simulink subsystem "Robot_Control_sub"  (R2026a)
settings: Solver=VariableStepAuto
undefined symbols (not defined in the file): Rebuilt_Hood_Servo_Pos_Max, Rebuilt_Hood_Servo_Pos_Min, TEST_Desired_Hood_Enable_OV, TEST_Desired_Hood_Pos_OV, TEST_Desired_Shooter_FF_DC_OV, TEST_Desired_Shooter_Speed_OV, TEST_Feeder_Motor_DC_OV, TEST_Intake_Arm_Motor_DC_OV, TEST_Intake_Roller_Motor_DC_OV, TEST_Output_Override_Flag, TEST_Transfer_Motor_DC_OV
libraries: Autonomous_lib x1, Disabled_lib x1, Controls_Components_lib x1, Teleop_lib x1, Test_lib x1
(part 2 of 2)

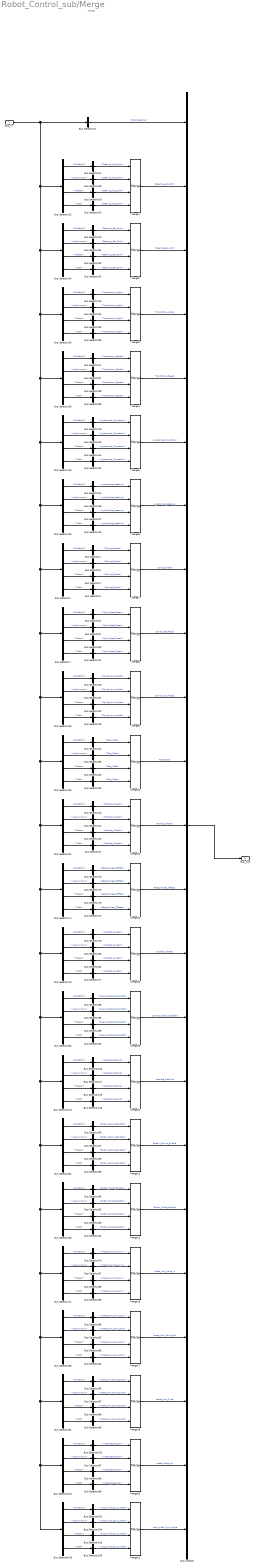
== system Robot_Control_sub/Merge ==
  note: Merge
  Bus_In : Inport
  Bus Creator : BusCreator  Inputs=23
  Bus Selector{1,3..5} (4 alike) : BusSelector  OutputSignals=Spline_Enable
  Bus Selector{9..10,22..23} (4 alike) : BusSelector  OutputSignals=Enable_Wheels
  Bus Selector{97..100} (4 alike) : BusSelector  OutputSignals=Intake_Roller_On
  Bus Selector{2,7,12,14,16,18,20..21,25,50,55,61,66,71,74,79,86,91,94,101,103,121} (22 alike) : BusSelector  OutputSignals=Disabled,Autonomous,Teleop,Test
  Bus Selector{102,104..106} (4 alike) : BusSelector  OutputSignals=Auto_Initial_Gyro_Angle
  Bus Selector{11,28..30} (4 alike) : BusSelector  OutputSignals=Steering_Abs_Cmd
  Bus Selector{117..120} (4 alike) : BusSelector  OutputSignals=Desired_Pipeline
  Bus Selector{13,31..33} (4 alike) : BusSelector  OutputSignals=Steering_Rel_Cmd
  Bus Selector{15,34..36} (4 alike) : BusSelector  OutputSignals=Translation_Angle
  Bus Selector{17,37..39} (4 alike) : BusSelector  OutputSignals=Translation_Speed
  Bus Selector{19,43..45} (4 alike) : BusSelector  OutputSignals=Is_Absolute_Translation
  Bus Selector{24,26..27,46} (4 alike) : BusSelector  OutputSignals=Is_Absolute_Steering
  Bus Selector{6,8,40..41} (4 alike) : BusSelector  OutputSignals=Spline_Ref_Poses
  Bus Selector{42,48..49,51} (4 alike) : BusSelector  OutputSignals=Spline_Num_Poses
  Bus Selector47 : BusSelector  OutputSignals=PreProcessing
  Bus Selector{52..54,56} (4 alike) : BusSelector  OutputSignals=Test_Mode
  Bus Selector{57..60} (4 alike) : BusSelector  OutputSignals=Button_Spinup_Enable
  Bus Selector{62..65} (4 alike) : BusSelector  OutputSignals=Button_Shoot_Enable
  Bus Selector{67..70} (4 alike) : BusSelector  OutputSignals=Intake_Arm_Move_In
  Bus Selector{72..73,75..76} (4 alike) : BusSelector  OutputSignals=Reset_Wheel_Offsets
  Bus Selector{77..78,80..81} (4 alike) : BusSelector  OutputSignals=Disable_Wheels
  Bus Selector{82..85} (4 alike) : BusSelector  OutputSignals=Intake_Arm_Move_Out
  Bus Selector{87..90} (4 alike) : BusSelector  OutputSignals=Intake_Arm_Move_Cycle
  Bus Selector{92..93,95..96} (4 alike) : BusSelector  OutputSignals=Swerve_Motors_Disabled
  Merge{1..21,24} (22 alike) : Merge  Inputs=4
  Bus_Out : Outport
  wires:
  Bus_In/1 -> Bus Selector47/1, Bus Selector12/1, Bus Selector14/1, Bus Selector16/1, Bus Selector18/1, Bus Selector20/1, Bus Selector25/1, Bus Selector21/1, Bus Selector74/1, Bus Selector121/1, Bus Selector61/1, Bus Selector66/1, Bus Selector71/1, Bus Selector86/1, Bus Selector91/1, Bus Selector101/1, Bus Selector103/1, Bus Selector94/1, Bus Selector79/1, Bus Selector55/1, Bus Selector50/1, Bus Selector7/1, Bus Selector2/1
  Merge21/1 -> Bus Creator/23  "Auto_Initial_Gyro_Angle"
  Bus Selector103/2 -> Bus Selector104/1  "<Autonomous>"
  Bus Selector105/1 -> Merge21/3  "<Auto_Initial_Gyro_Angle>"
  Bus Selector103/3 -> Bus Selector105/1  "<Teleop>"
  Bus Selector102/1 -> Merge21/1  "<Auto_Initial_Gyro_Angle>"
  Bus Selector104/1 -> Merge21/2  "<Auto_Initial_Gyro_Angle>"
  Bus Selector103/1 -> Bus Selector102/1  "<Disabled>"
  Bus Selector103/4 -> Bus Selector106/1  "<Test>"
  Bus Selector106/1 -> Merge21/4  "<Auto_Initial_Gyro_Angle>"
  Bus Selector99/1 -> Merge20/4  "<Intake_Roller_On>"
  Bus Selector98/1 -> Merge20/3  "<Intake_Roller_On>"
  Bus Selector97/1 -> Merge20/2  "<Intake_Roller_On>"
  Bus Selector89/1 -> Merge18/4  "<Intake_Arm_Move_Cycle>"
  Bus Selector88/1 -> Merge18/3  "<Intake_Arm_Move_Cycle>"
  Bus Selector87/1 -> Merge18/2  "<Intake_Arm_Move_Cycle>"
  Bus Selector84/1 -> Merge17/4  "<Intake_Arm_Move_Out>"
  Bus Selector83/1 -> Merge17/3  "<Intake_Arm_Move_Out>"
  Bus Selector82/1 -> Merge17/2  "<Intake_Arm_Move_Out>"
  Bus Selector69/1 -> Merge13/4  "<Intake_Arm_Move_In>"
  Bus Selector68/1 -> Merge13/3  "<Intake_Arm_Move_In>"
  Bus Selector67/1 -> Merge13/2  "<Intake_Arm_Move_In>"
  Merge20/1 -> Bus Creator/22  "Intake_Roller_On"
  Bus Selector101/1 -> Bus Selector100/1  "<Disabled>"
  Bus Selector101/3 -> Bus Selector98/1  "<Teleop>"
  Bus Selector100/1 -> Merge20/1  "<Intake_Roller_On>"
  Bus Selector101/2 -> Bus Selector97/1  "<Autonomous>"
  Bus Selector101/4 -> Bus Selector99/1  "<Test>"
  Merge18/1 -> Bus Creator/21  "Intake_Arm_Cycle"
  Bus Selector91/4 -> Bus Selector89/1  "<Test>"
  Bus Selector91/2 -> Bus Selector87/1  "<Autonomous>"
  Bus Selector90/1 -> Merge18/1  "<Intake_Arm_Move_Cycle>"
  Bus Selector91/3 -> Bus Selector88/1  "<Teleop>"
  Bus Selector91/1 -> Bus Selector90/1  "<Disabled>"
  Merge17/1 -> Bus Creator/20  "Intake_Arm_Move_Out"
  Bus Selector86/1 -> Bus Selector85/1  "<Disabled>"
  Bus Selector86/3 -> Bus Selector83/1  "<Teleop>"
  Bus Selector85/1 -> Merge17/1  "<Intake_Arm_Move_Out>"
  Bus Selector86/2 -> Bus Selector82/1  "<Autonomous>"
  Bus Selector86/4 -> Bus Selector84/1  "<Test>"
  Merge13/1 -> Bus Creator/19  "Intake_Arm_Move_In"
  Bus Selector71/4 -> Bus Selector69/1  "<Test>"
  Bus Selector70/1 -> Merge13/1  "<Intake_Arm_Move_In>"
  Bus Selector71/1 -> Bus Selector70/1  "<Disabled>"
  Bus Selector71/3 -> Bus Selector68/1  "<Teleop>"
  Bus Selector71/2 -> Bus Selector67/1  "<Autonomous>"
  Bus Selector64/1 -> Merge12/4  "<Button_Shoot_Enable>"
  Bus Selector63/1 -> Merge12/3  "<Button_Shoot_Enable>"
  Bus Selector62/1 -> Merge12/2  "<Button_Shoot_Enable>"
  Bus Selector59/1 -> Merge11/4  "<Button_Spinup_Enable>"
  Bus Selector58/1 -> Merge11/3  "<Button_Spinup_Enable>"
  Bus Selector57/1 -> Merge11/2  "<Button_Spinup_Enable>"
  Bus Selector65/1 -> Merge12/1  "<Button_Shoot_Enable>"
  Bus Selector66/2 -> Bus Selector62/1  "<Autonomous>"
  Bus Selector66/3 -> Bus Selector63/1  "<Teleop>"
  Bus Selector66/1 -> Bus Selector65/1  "<Disabled>"
  Bus Selector66/4 -> Bus Selector64/1  "<Test>"
  Bus Selector61/2 -> Bus Selector57/1  "<Autonomous>"
  Bus Selector60/1 -> Merge11/1  "<Button_Spinup_Enable>"
  Bus Selector61/1 -> Bus Selector60/1  "<Disabled>"
  Bus Selector61/4 -> Bus Selector59/1  "<Test>"
  Bus Selector61/3 -> Bus Selector58/1  "<Teleop>"
  Merge12/1 -> Bus Creator/18  "Button_Shoot_Enable"
  Merge11/1 -> Bus Creator/17  "Button_Spinup_Enable"
  Bus Selector47/1 -> Bus Creator/1  "<PreProcessing>"
  Merge24/1 -> Bus Creator/16  "Desired_Pipeline"
  Bus Selector119/1 -> Merge24/3  "<Desired_Pipeline>"
  Bus Selector118/1 -> Merge24/4  "<Desired_Pipeline>"
  Bus Selector117/1 -> Merge24/2  "<Desired_Pipeline>"
  Bus Selector120/1 -> Merge24/1  "<Desired_Pipeline>"
  Bus Selector121/2 -> Bus Selector117/1  "<Autonomous>"
  Bus Selector121/1 -> Bus Selector120/1  "<Disabled>"
  Bus Selector121/3 -> Bus Selector119/1  "<Teleop>"
  Bus Selector121/4 -> Bus Selector118/1  "<Test>"
  Merge19/1 -> Bus Creator/15  "Swerve_Motors_Disabled"
  Merge16/1 -> Bus Creator/14  "Disable_Wheels"
  Merge15/1 -> Bus Creator/13  "Reset_Wheel_Offsets"
  Merge14/1 -> Bus Creator/12  "Enable_Wheels"
  Bus Creator/1 -> Bus_Out/1
  Bus Selector21/4 -> Bus Selector9/1  "<Test>"
  Bus Selector9/1 -> Merge14/4  "<Enable_Wheels>"
  Bus Selector21/3 -> Bus Selector23/1  "<Teleop>"
  Bus Selector21/2 -> Bus Selector22/1  "<Autonomous>"
  Bus Selector10/1 -> Merge14/1  "<Enable_Wheels>"
  Bus Selector22/1 -> Merge14/2  "<Enable_Wheels>"
  Bus Selector21/1 -> Bus Selector10/1  "<Disabled>"
  Bus Selector23/1 -> Merge14/3  "<Enable_Wheels>"
  Bus Selector94/4 -> Bus Selector92/1  "<Test>"
  Bus Selector93/1 -> Merge19/1  "<Swerve_Motors_Disabled>"
  Bus Selector94/2 -> Bus Selector95/1  "<Autonomous>"
  Bus Selector92/1 -> Merge19/4  "<Swerve_Motors_Disabled>"
  Bus Selector94/3 -> Bus Selector96/1  "<Teleop>"
  Bus Selector94/1 -> Bus Selector93/1  "<Disabled>"
  Bus Selector96/1 -> Merge19/3  "<Swerve_Motors_Disabled>"
  Bus Selector95/1 -> Merge19/2  "<Swerve_Motors_Disabled>"
  Bus Selector81/1 -> Merge16/3  "<Disable_Wheels>"
  Bus Selector79/4 -> Bus Selector77/1  "<Test>"
  Bus Selector79/1 -> Bus Selector78/1  "<Disabled>"
  Bus Selector79/3 -> Bus Selector81/1  "<Teleop>"
  Bus Selector79/2 -> Bus Selector80/1  "<Autonomous>"
  Bus Selector77/1 -> Merge16/4  "<Disable_Wheels>"
  Bus Selector78/1 -> Merge16/1  "<Disable_Wheels>"
  Bus Selector80/1 -> Merge16/2  "<Disable_Wheels>"
  Bus Selector74/4 -> Bus Selector72/1  "<Test>"
  Bus Selector74/2 -> Bus Selector75/1  "<Autonomous>"
  Bus Selector74/1 -> Bus Selector73/1  "<Disabled>"
  Bus Selector75/1 -> Merge15/2  "<Reset_Wheel_Offsets>"
  Bus Selector76/1 -> Merge15/3  "<Reset_Wheel_Offsets>"
  Bus Selector74/3 -> Bus Selector76/1  "<Teleop>"
  Bus Selector72/1 -> Merge15/4  "<Reset_Wheel_Offsets>"
  Bus Selector73/1 -> Merge15/1  "<Reset_Wheel_Offsets>"
  Merge10/1 -> Bus Creator/11  "Test_Mode"
  Bus Selector55/2 -> Bus Selector56/1  "<Autonomous>"
  Bus Selector53/1 -> Merge10/4  "<Test_Mode>"
  Bus Selector54/1 -> Merge10/1  "<Test_Mode>"
  Bus Selector55/1 -> Bus Selector54/1  "<Disabled>"
  Bus Selector55/4 -> Bus Selector53/1  "<Test>"
  Bus Selector56/1 -> Merge10/2  "<Test_Mode>"
  Bus Selector52/1 -> Merge10/3  "<Test_Mode>"
  Bus Selector55/3 -> Bus Selector52/1  "<Teleop>"
  Merge9/1 -> Bus Creator/10  "Spline_Num_Poses"
  Bus Selector48/1 -> Merge9/4  "<Spline_Num_Poses>"
  Bus Selector50/1 -> Bus Selector49/1  "<Disabled>"
  Bus Selector42/1 -> Merge9/3  "<Spline_Num_Poses>"
  Bus Selector49/1 -> Merge9/1  "<Spline_Num_Poses>"
  Bus Selector51/1 -> Merge9/2  "<Spline_Num_Poses>"
  Bus Selector50/4 -> Bus Selector48/1  "<Test>"
  Bus Selector50/3 -> Bus Selector42/1  "<Teleop>"
  Bus Selector50/2 -> Bus Selector51/1  "<Autonomous>"
  Merge8/1 -> Bus Creator/9  "Spline_Ref_Poses"
  Bus Selector7/2 -> Bus Selector8/1  "<Autonomous>"
  Bus Selector7/3 -> Bus Selector40/1  "<Teleop>"
  Bus Selector7/4 -> Bus Selector41/1  "<Test>"
  Bus Selector8/1 -> Merge8/2  "<Spline_Ref_Poses>"
  Bus Selector6/1 -> Merge8/1  "<Spline_Ref_Poses>"
  Bus Selector40/1 -> Merge8/3  "<Spline_Ref_Poses>"
  Bus Selector7/1 -> Bus Selector6/1  "<Disabled>"
  Bus Selector41/1 -> Merge8/4  "<Spline_Ref_Poses>"
  Merge7/1 -> Bus Creator/8  "Spline_Enable"
  Bus Selector5/1 -> Merge7/4  "<Spline_Enable>"
  Bus Selector2/1 -> Bus Selector1/1  "<Disabled>"
  Bus Selector4/1 -> Merge7/3  "<Spline_Enable>"
  Bus Selector1/1 -> Merge7/1  "<Spline_Enable>"
  Bus Selector3/1 -> Merge7/2  "<Spline_Enable>"
  Bus Selector2/4 -> Bus Selector5/1  "<Test>"
  Bus Selector2/3 -> Bus Selector4/1  "<Teleop>"
  Bus Selector2/2 -> Bus Selector3/1  "<Autonomous>"
  Bus Selector29/1 -> Merge1/3  "<Steering_Abs_Cmd>"
  Bus Selector25/2 -> Bus Selector26/1  "<Autonomous>"
  Bus Selector25/3 -> Bus Selector27/1  "<Teleop>"
  Bus Selector14/3 -> Bus Selector32/1  "<Teleop>"
  Bus Selector16/3 -> Bus Selector35/1  "<Teleop>"
  Bus Selector16/4 -> Bus Selector36/1  "<Test>"
  Bus Selector20/1 -> Bus Selector19/1  "<Disabled>"
  Merge1/1 -> Bus Creator/2  "Steering_Abs_Cmd"
  Bus Selector34/1 -> Merge3/2  "<Translation_Angle>"
  Bus Selector17/1 -> Merge4/1  "<Translation_Speed>"
  Bus Selector15/1 -> Merge3/1  "<Translation_Angle>"
  Bus Selector20/2 -> Bus Selector43/1  "<Autonomous>"
  Bus Selector14/1 -> Bus Selector13/1  "<Disabled>"
  Bus Selector20/4 -> Bus Selector45/1  "<Test>"
  Merge5/1 -> Bus Creator/6  "Is_Absolute_Translation"
  Bus Selector36/1 -> Merge3/4  "<Translation_Angle>"
  Bus Selector12/1 -> Bus Selector11/1  "<Disabled>"
  Bus Selector16/2 -> Bus Selector34/1  "<Autonomous>"
  Bus Selector37/1 -> Merge4/2  "<Translation_Speed>"
  Bus Selector25/4 -> Bus Selector46/1  "<Test>"
  Bus Selector18/3 -> Bus Selector38/1  "<Teleop>"
  Bus Selector20/3 -> Bus Selector44/1  "<Teleop>"
  Bus Selector39/1 -> Merge4/4  "<Translation_Speed>"
  Bus Selector16/1 -> Bus Selector15/1  "<Disabled>"
  Bus Selector13/1 -> Merge2/1  "<Steering_Rel_Cmd>"
  Bus Selector30/1 -> Merge1/4  "<Steering_Abs_Cmd>"
  Bus Selector26/1 -> Merge6/2  "<Is_Absolute_Steering>"
  Merge6/1 -> Bus Creator/7  "Is_Absolute_Steering"
  Bus Selector18/1 -> Bus Selector17/1  "<Disabled>"
  Bus Selector45/1 -> Merge5/4  "<Is_Absolute_Translation>"
  Bus Selector12/3 -> Bus Selector29/1  "<Teleop>"
  Bus Selector18/2 -> Bus Selector37/1  "<Autonomous>"
  Bus Selector43/1 -> Merge5/2  "<Is_Absolute_Translation>"
  Bus Selector19/1 -> Merge5/1  "<Is_Absolute_Translation>"
  Bus Selector35/1 -> Merge3/3  "<Translation_Angle>"
  Merge3/1 -> Bus Creator/4  "Translation_Angle"
  Bus Selector28/1 -> Merge1/2  "<Steering_Abs_Cmd>"
  Bus Selector14/2 -> Bus Selector31/1  "<Autonomous>"
  Bus Selector32/1 -> Merge2/3  "<Steering_Rel_Cmd>"
  Merge4/1 -> Bus Creator/5  "Translation_Speed"
  Bus Selector12/2 -> Bus Selector28/1  "<Autonomous>"
  Bus Selector14/4 -> Bus Selector33/1  "<Test>"
  Bus Selector44/1 -> Merge5/3  "<Is_Absolute_Translation>"
  Bus Selector24/1 -> Merge6/1  "<Is_Absolute_Steering>"
  Bus Selector11/1 -> Merge1/1  "<Steering_Abs_Cmd>"
  Bus Selector31/1 -> Merge2/2  "<Steering_Rel_Cmd>"
  Bus Selector27/1 -> Merge6/3  "<Is_Absolute_Steering>"
  Bus Selector25/1 -> Bus Selector24/1  "<Disabled>"
  Bus Selector18/4 -> Bus Selector39/1  "<Test>"
  Bus Selector46/1 -> Merge6/4  "<Is_Absolute_Steering>"
  Bus Selector38/1 -> Merge4/3  "<Translation_Speed>"
  Bus Selector33/1 -> Merge2/4  "<Steering_Rel_Cmd>"
  Bus Selector12/4 -> Bus Selector30/1  "<Test>"
  Merge2/1 -> Bus Creator/3  "Steering_Rel_Cmd"

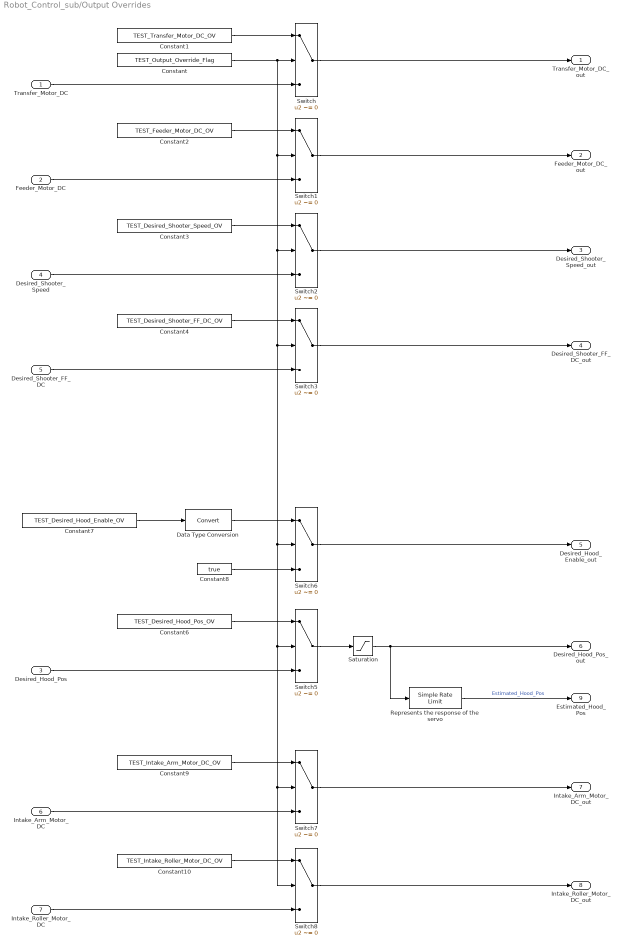
== system Robot_Control_sub/Output Overrides ==
  Transfer_Motor_DC : Inport
  Feeder_Motor_DC : Inport  Port=2
  Desired_Hood_Pos : Inport  Port=3
  Desired_Shooter_Speed : Inport  Port=4
  Desired_Shooter_FF_DC : Inport  Port=5
  Intake_Arm_Motor_DC : Inport  Port=6
  Intake_Roller_Motor_DC : Inport  Port=7
  Constant : Constant  Value=TEST_Output_Override_Flag
  Constant1 : Constant  Value=TEST_Transfer_Motor_DC_OV
  Constant10 : Constant  Value=TEST_Intake_Roller_Motor_DC_OV
  Constant2 : Constant  Value=TEST_Feeder_Motor_DC_OV
  Constant3 : Constant  Value=TEST_Desired_Shooter_Speed_OV
  Constant4 : Constant  Value=TEST_Desired_Shooter_FF_DC_OV
  Constant6 : Constant  Value=TEST_Desired_Hood_Pos_OV
  Constant7 : Constant  Value=TEST_Desired_Hood_Enable_OV
  Constant8 : Constant  Value=true
  Constant9 : Constant  Value=TEST_Intake_Arm_Motor_DC_OV
  Data Type Conversion : DataTypeConversion  SaturateOnIntegerOverflow=off  RndMeth=Floor
  Represents the response of the servo : Controls_Components_lib/Simple Rate Limit  Rate_Limit_Inc=Rebuilt_Hood_Servo_Rate_Limit_Inc  Rate_Limit_Dec=Rebuilt_Hood_Servo_Rate_Limit_Dec
  Saturation : Saturate  UpperLimit=Rebuilt_Hood_Servo_Pos_Max  LowerLimit=Rebuilt_Hood_Servo_Pos_Min
  Switch{,1..3,5..8} (8 alike) : Switch  Criteria=u2 ~= 0  SaturateOnIntegerOverflow=off  InputSameDT=off
  Transfer_Motor_DC_out : Outport
  Feeder_Motor_DC_out : Outport  Port=2
  Desired_Shooter_Speed_out : Outport  Port=3
  Desired_Shooter_FF_DC_out : Outport  Port=4
  Desired_Hood_Enable_out : Outport  Port=5
  Desired_Hood_Pos_out : Outport  Port=6
  Intake_Arm_Motor_DC_out : Outport  Port=7
  Intake_Roller_Motor_DC_out : Outport  Port=8
  Estimated_Hood_Pos : Outport  Port=9
  wires:
  Switch8/1 -> Intake_Roller_Motor_DC_out/1
  Switch7/1 -> Intake_Arm_Motor_DC_out/1
  Constant10/1 -> Switch8/1
  Constant9/1 -> Switch7/1
  Intake_Roller_Motor_DC/1 -> Switch8/3
  Intake_Arm_Motor_DC/1 -> Switch7/3
  Data Type Conversion/1 -> Switch6/1
  Represents the response of the servo/1 -> Estimated_Hood_Pos/1  "Estimated_Hood_Pos"
  Saturation/1 -> Desired_Hood_Pos_out/1, Represents the response of the servo/1
  Constant8/1 -> Switch6/3
  Switch6/1 -> Desired_Hood_Enable_out/1
  Constant7/1 -> Data Type Conversion/1
  Switch5/1 -> Saturation/1
  Switch3/1 -> Desired_Shooter_FF_DC_out/1
  Switch2/1 -> Desired_Shooter_Speed_out/1
  Switch1/1 -> Feeder_Motor_DC_out/1
  Switch/1 -> Transfer_Motor_DC_out/1
  Desired_Hood_Pos/1 -> Switch5/3
  Constant6/1 -> Switch5/1
  Desired_Shooter_FF_DC/1 -> Switch3/3
  Desired_Shooter_Speed/1 -> Switch2/3
  Feeder_Motor_DC/1 -> Switch1/3
  Constant4/1 -> Switch3/1
  Constant3/1 -> Switch2/1
  Constant2/1 -> Switch1/1
  Constant1/1 -> Switch/1
  Transfer_Motor_DC/1 -> Switch/3
  Constant/1 -> Switch/2, Switch1/2, Switch2/2, Switch3/2, Switch5/2, Switch7/2, Switch8/2, Switch6/2

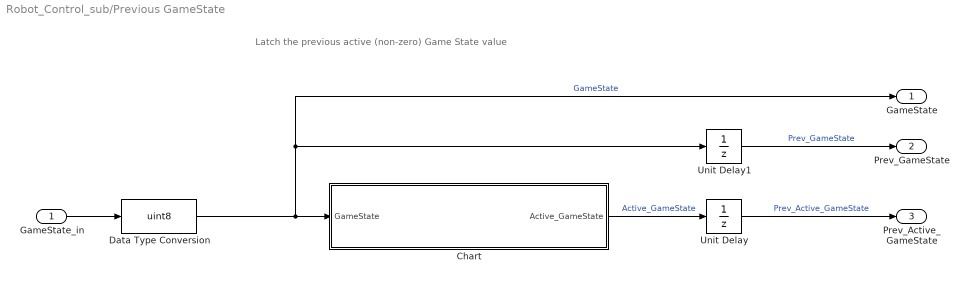
== system Robot_Control_sub/Previous GameState ==
  note: Latch the previous active (non-zero) Game State value
  GameState_in : Inport
  Chart : Stateflow chart  TreatAsAtomicUnit=on
  Data Type Conversion : DataTypeConversion  OutDataTypeStr=uint8  SaturateOnIntegerOverflow=off  RndMeth=Floor
  Unit Delay : UnitDelay  SampleTime=-1
  Unit Delay1 : UnitDelay  SampleTime=-1
  GameState : Outport
  Prev_GameState : Outport  Port=2
  Prev_Active_GameState : Outport  Port=3
  wires:
  Unit Delay1/1 -> Prev_GameState/1  "Prev_GameState"
  Chart/1(Active_GameState) -> Unit Delay/1  "Active_GameState"
  Data Type Conversion/1 -> Chart/1(GameState), GameState/1, Unit Delay1/1  "GameState"
  Unit Delay/1 -> Prev_Active_GameState/1  "Prev_Active_GameState"
  GameState_in/1 -> Data Type Conversion/1

== stateflow chart Robot_Control_sub/Previous GameState/Chart ==
  state Disabled
  state Not_Disabled
    en: Active_GameState = GameState;
    du: Active_GameState = GameState;
  (default) -> Disabled : {Active_GameState = 0}
  Disabled -> Not_Disabled : [GameState ~= 0]
  Not_Disabled -> Disabled : [GameState == 0]
  data: GameState input; Active_GameState output
